simulink model "PAC_autotuning_online_v01"  (R2025a)
settings: Solver=VariableStepAuto  StartTime=0.0  StopTime=inf  RelTol=1e-3
undefined symbols (not defined in the file or in its folder): National_Instruments, PCI
libraries: sldrtlib x3, simulink x1
(part 2 of 2)

== matlab function PAC_autotuning_online_v01/Online zero command confirmation ==
  settings: updateMethod=DISCRETE  sampleTime=0.05
  data: t input; ready output; done input; pressure input size=[3 1]
function ready=stopReady(t,done,pressure)
%#codegen
ready=pacOnlineStopReady(t,done,pressure);
end

== matlab function PAC_autotuning_online_v01/PAC ==
  settings: updateMethod=DISCRETE  sampleTime=0.05
  data: measured input; desired input; gravity_arm input; measurementValid input; baseValid input; measurementTime_s input; t input; pressureCommand_bar output double; tauRequested_N output double; tauEquivalent_N output double; allocationResidual_N output; s_mPerS output; inertiaForce_N output; coriolisForce_N output; dampingForce_N output; staticForce_N output; feedbackForce_N output; modelValid output boolean; limited output boolean; enablePressure input; status output uint8 size=1; allAboveActivation output boolean; anchorReady output boolean; forceBias_N output; tauBlended_N output; lambda input; dampingGain input; enableAdaptation input; stiffnessEstimate_NPerM output; dampingEstimate_NsPerM output; hysteresisForce_N output; adaptiveBias_N output; parameterEstimate output; historyState output; adaptationActive output; parameterAtBound output; adaptiveForce_N output; enableCommonPressureAdaptation input; adaptationGamma input; parameterScale input; parameterMaxRate input; parameterLower input; parameterUpper input; parameterInitial input; adaptationOptions input; historyOptions input; pressureOptions input; supervisorOptions input; commonPressure_bar output; commonPressureShift_bar output; freezeHysteresisWeights input
function [pressureCommand_bar,tauRequested_N,tauEquivalent_N, ...
 allocationResidual_N,s_mPerS,inertiaForce_N,coriolisForce_N, ...
 dampingForce_N,staticForce_N,feedbackForce_N,modelValid,limited, ...
 status,allAboveActivation,anchorReady,forceBias_N,tauBlended_N, ...
 stiffnessEstimate_NPerM,dampingEstimate_NsPerM,hysteresisForce_N, ...
 adaptiveBias_N,parameterEstimate,historyState,adaptationActive, ...
 parameterAtBound,adaptiveForce_N,commonPressure_bar,commonPressureShift_bar] = pacAdaptiveTunableBlock( ...
 measured,desired,gravity_arm,measurementValid,baseValid,measurementTime_s, ...
 t,enablePressure,lambda,dampingGain,enableAdaptation, ...
 enableCommonPressureAdaptation,adaptationGamma,parameterScale,parameterMaxRate, ...
 parameterLower,parameterUpper,parameterInitial,adaptationOptions, ...
 historyOptions,pressureOptions,supervisorOptions,freezeHysteresisWeights)
%#codegen
% Paste into a separate controller block; Discrete .05 s. Existing first 11 inputs
% and first 26 outputs preserved. Tuning port sizes: see TUNABLE_BLOCK.md.
% Estimates correspond to force evaluation; updates take effect NEXT sample.
% Append Boolean freezeHysteresisWeights: true holds h1/h2/h3 only.
% History states keep evolving; false resumes normal gated adaptation.
if nargin<23
 freezeHysteresisWeights=false;
end
[cfg,pc]=pacTuningConfig(adaptationGamma,parameterScale,parameterMaxRate, ...
 parameterLower,parameterUpper,parameterInitial,adaptationOptions, ...
 historyOptions,pressureOptions,supervisorOptions);
if freezeHysteresisWeights
 cfg.gamma(6:8)=0;
end
pc.enableCommonAdaptation=logical(enableCommonPressureAdaptation);
persistent ps as
if isempty(ps)
 ps=pacPressureInitialState();as=pacAdaptiveInitialState();as.theta=cfg.initial;
end
good=measurementValid && baseValid && isfinite(measurementTime_s) && ...
 isfinite(t) && measurementTime_s<=t+1e-9 && ...
 t-measurementTime_s<=pc.maxSampleAge_s+1e-9;
dt=0;
if good && measurementTime_s>as.lastSample
 if as.lastSample>=0,dt=measurementTime_s-as.lastSample;end
 if all(isfinite(measured(:))) && ~ps.fault
  as.z=pacAdaptiveHistory(as.z,measured(3:4),dt,cfg);
 end
 as.lastSample=measurementTime_s;
end
[tauRequested_N,s_mPerS,Y,inertiaForce_N,coriolisForce_N, ...
 dampingForce_N,staticForce_N,feedbackForce_N,hysteresisForce_N, ...
 adaptiveBias_N,stiffnessEstimate_NPerM,dampingEstimate_NsPerM,modelValid]= ...
 pacAdaptiveForce(measured,desired,gravity_arm,lambda,dampingGain,as,good);
% Capture nominal static+history+bias consistently with current model at trim.
[pressureCommand_bar,tauEquivalent_N,allocationResidual_N,limited,status, ...
 allAboveActivation,tauBlended_N,ps]=pacPressureStep(tauRequested_N, ...
 staticForce_N+hysteresisForce_N+adaptiveBias_N,measured(3:4),modelValid, ...
 measurementTime_s,t,enablePressure,pc,ps);
commonPressure_bar=mean(pressureCommand_bar);
commonPressureShift_bar=commonPressure_bar-pc.common_bar;
anchorReady=ps.anchorReady;forceBias_N=ps.forceBias;
parameterEstimate=as.theta;historyState=as.z;
[p,~,~]=pacNominalParameters(gravity_arm);
q=measured(1:2);v=desired(3:4)-lambda(:).*(q-desired(1:2));
adaptiveForce_N=(stiffnessEstimate_NPerM-p.K)*q+ ...
 (dampingEstimate_NsPerM-p.D)*v+hysteresisForce_N+adaptiveBias_N;
allow=enableAdaptation && good && modelValid && status==uint8(3) && ...
 ~limited && all(isfinite(allocationResidual_N)) && ...
 norm(allocationResidual_N)<=cfg.residualTolerance_N;
[as,adaptationActive,parameterAtBound]=pacAdaptiveUpdate(as,Y,s_mPerS,dt,allow,cfg);
end
